simulink model "NBMS_SoC"  (R2026b)
settings: Solver=FixedStepDiscrete  StopTime=25  FixedStep=0.1
undefined symbols (not defined in the file): BMS_BattSoCDerate_E, BMS_BattTempDerate_E, BMS_MODE_E, CAL_15_SOC_WRN_RVL_THRSH, CAL_15_SOC_WRN_THRSH, CAL_DCHRG_END_THRSH, CAL_DOD, CAL_DOD_MAX_THRSH, CAL_DOD_MIN_THRSH, CAL_ENABLE_SOC_WARN_15, CAL_ENABLE_SOC_WARN_20, CAL_GOLDEN_CHARGE, CAL_GOLDEN_DC, CAL_LOW_SOC_RVL_THRSH, CAL_LOW_SOC_THRSH, CAL_NOMINAL_VOLTAGE, CAL_SOC_WRN_RVL_THRSH, CAL_SOC_WRN_THRSH, CAL_SOH_Enable, Charger_Mode_Req_E, DiscIntNeverNeededParam, OBC_E, VDU_MACHINE_STS_E, X_DCIR_CHG, X_DCIR_DISCH, Y_DCIR_CHG, Y_DCIR_DISCH
libraries: simulink x110, simulink_extras x6, sl_discontinuities x3
(part 1 of 3)
settings Model: Creator=hp  LastModifiedBy=rathi
settings OptimizationCC: DefaultParameterBehavior=Inlined  DifferentSizesBufferReuse=on  EfficientTunableParamExpr=on  EnhancedBackFolding=on  OptimizationCustomize=off  OptimizeBlockOrder=speed  PassReuseOutputArgsAs=Individual arguments  RemoveInternalMemoryZeroInit=on  RemoveRootLevelIOMemoryZeroInit=on
settings DebuggingCC: ParameterTunabilityLossMsg=error
settings SFSimCC: MATLABDynamicMemAlloc=off
settings RTWCC: Description=Embedded Coder  GenCodeOnly=on  PackageGeneratedCodeAndArtifacts=on  SystemTargetFile=ert.tlc  TemplateMakefile=ert_default_tmf
settings CodeAppCC: ForceParamTrailComments=on  IgnoreCustomStorageClasses=off  InsertBlockDesc=on  OperatorAnnotations=on  SFDataObjDesc=on  SimulinkDataObjDesc=on
settings ERTTargetCC: DynamicArrayContainerType=coder::array  GenerateSampleERTMain=on
settings ConfigComp: DVDefectChecker=on  DVDetectOutOfBounds=on  DVHarnessSource=Signal Editor  DVModelReferenceHarness=on  DVTestSuiteOptimization=Auto

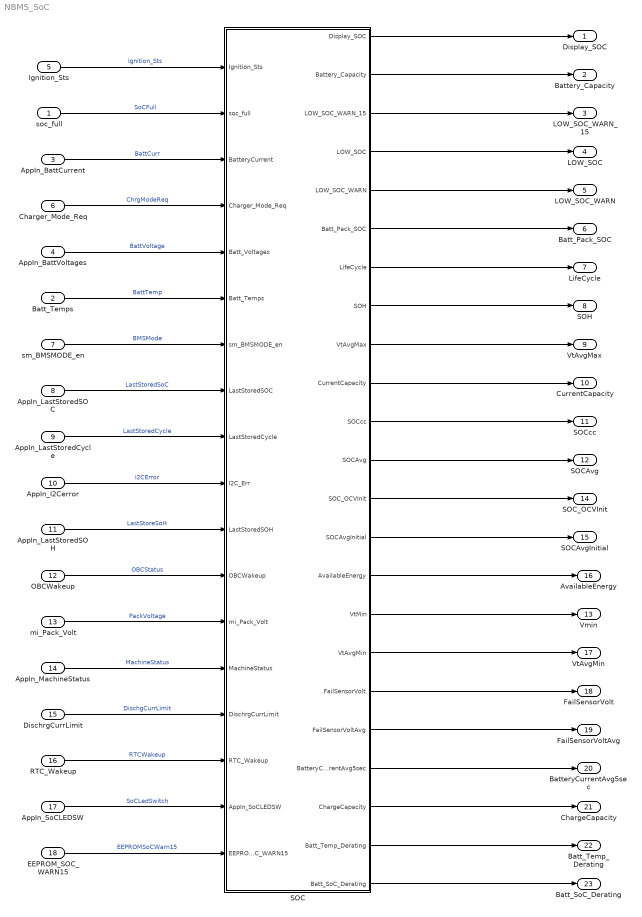
== system NBMS_SoC ==
  soc_full : Inport  OutDataTypeStr=uint8
  Batt_Temps : Inport  Port=2  OutDataTypeStr=double
  AppIn_BattCurrent : Inport  Port=3
  AppIn_BattVoltages : Inport  Port=4  OutDataTypeStr=double  PortDimensions=[20,1]
  Ignition_Sts : Inport  Port=5  OutDataTypeStr=boolean
  Charger_Mode_Req : Inport  Port=6  OutDataTypeStr=Enum:Charger_Mode_Req_E
  sm_BMSMODE_en : Inport  Port=7  OutDataTypeStr=Enum: BMS_MODE_E
  AppIn_LastStoredSOC : Inport  Port=8  OutDataTypeStr=double
  AppIn_LastStoredCycle : Inport  Port=9  OutDataTypeStr=double
  AppIn_I2Cerror : Inport  Port=10  OutDataTypeStr=boolean
  AppIn_LastStoredSOH : Inport  Port=11  OutDataTypeStr=double
  OBCWakeup : Inport  Port=12  OutDataTypeStr=Enum: OBC_E
  mi_Pack_Volt : Inport  Port=13  OutDataTypeStr=double
  AppIn_MachineStatus : Inport  Port=14  OutDataTypeStr=Enum: VDU_MACHINE_STS_E
  DischrgCurrLimit : Inport  Port=15
  RTC_Wakeup : Inport  Port=16  OutDataTypeStr=boolean
  AppIn_SoCLEDSW : Inport  Port=17  OutDataTypeStr=boolean
  EEPROM_SOC_WARN15 : Inport  Port=18  OutDataTypeStr=boolean
  SOC : Subsystem
  Display_SOC : Outport  OutDataTypeStr=uint8
  Battery_Capacity : Outport  Port=2
  LOW_SOC_WARN_15 : Outport  Port=3  OutDataTypeStr=boolean
  LOW_SOC : Outport  Port=4  OutDataTypeStr=boolean
  LOW_SOC_WARN : Outport  Port=5  OutDataTypeStr=boolean
  Batt_Pack_SOC : Outport  Port=6
  LifeCycle : Outport  Port=7  OutDataTypeStr=double
  SOH : Outport  Port=8  OutDataTypeStr=double
  VtAvgMax : Outport  Port=9  OutDataTypeStr=fixdt(1,16,0.001,0)
  CurrentCapacity : Outport  Port=10  OutDataTypeStr=double
  SOCcc : Outport  Port=11  OutDataTypeStr=fixdt(0,16,0.01,0)
  SOCAvg : Outport  Port=12  OutDataTypeStr=fixdt(0,16,0.01,0)
  Vmin : Outport  Port=13  OutDataTypeStr=fixdt(1,16,0.001,0)
  SOC_OCVInit : Outport  Port=14  OutDataTypeStr=double
  SOCAvgInitial : Outport  Port=15  OutDataTypeStr=double
  AvailableEnergy : Outport  Port=16  OutDataTypeStr=double
  VtAvgMin : Outport  Port=17
  FailSensorVolt : Outport  Port=18  OutputWhenDisabled=reset  InitialOutput=5
  FailSensorVoltAvg : Outport  Port=19  OutputWhenDisabled=reset  InitialOutput=5
  BatteryCurrentAvg5sec : Outport  Port=20  OutDataTypeStr=fixdt(1,16,0.01,0)
  ChargeCapacity : Outport  Port=21  OutDataTypeStr=double
  Batt_Temp_Derating : Outport  Port=22  OutDataTypeStr=Enum: BMS_BattTempDerate_E
  Batt_SoC_Derating : Outport  Port=23  OutDataTypeStr=Enum: BMS_BattSoCDerate_E
  wires:
  SOC/5(" LOW_SOC_WARN") -> LOW_SOC_WARN/1
  SOC/13(SOC_OCVInit) -> SOC_OCVInit/1
  SOC/17(VtAvgMin) -> VtAvgMin/1
  SOC/9(VtAvgMax) -> VtAvgMax/1
  SOC/14(SOCAvgInitial) -> SOCAvgInitial/1
  SOC/21(ChargeCapacity) -> ChargeCapacity/1
  SOC/1(Display_SOC) -> Display_SOC/1
  SOC/15(AvailableEnergy) -> AvailableEnergy/1
  AppIn_LastStoredCycle/1 -> SOC/9(LastStoredCycle)  "LastStoredCycle"
  SOC/11(SOCcc) -> SOCcc/1
  SOC/8(SOH) -> SOH/1
  OBCWakeup/1 -> SOC/12(OBCWakeup)  "OBCStatus"
  SOC/16(VtMin) -> Vmin/1
  SOC/10(CurrentCapacity) -> CurrentCapacity/1
  SOC/6(Batt_Pack_SOC) -> Batt_Pack_SOC/1
  AppIn_BattVoltages/1 -> SOC/5(Batt_Voltages)  "BattVoltage"
  SOC/12(SOCAvg) -> SOCAvg/1
  SOC/20(BatteryCurrentAvg5sec) -> BatteryCurrentAvg5sec/1
  AppIn_LastStoredSOH/1 -> SOC/11(LastStoredSOH)  "LastStoreSoH"
  SOC/7(LifeCycle) -> LifeCycle/1
  SOC/3(" LOW_SOC_WARN_15") -> LOW_SOC_WARN_15/1
  SOC/2(Battery_Capacity) -> Battery_Capacity/1
  mi_Pack_Volt/1 -> SOC/13(mi_Pack_Volt)  "PackVoltage"
  DischrgCurrLimit/1 -> SOC/15(DischrgCurrLimit)  "DischgCurrLimit"
  SOC/4(" LOW_SOC") -> LOW_SOC/1
  SOC/19(FailSensorVoltAvg) -> FailSensorVoltAvg/1
  Charger_Mode_Req/1 -> SOC/4(Charger_Mode_Req)  "ChrgModeReq"
  sm_BMSMODE_en/1 -> SOC/7(sm_BMSMODE_en)  "BMSMode"
  Batt_Temps/1 -> SOC/6(Batt_Temps)  "BattTemp"
  AppIn_MachineStatus/1 -> SOC/14(MachineStatus)  "MachineStatus"
  SOC/18(FailSensorVolt) -> FailSensorVolt/1
  AppIn_I2Cerror/1 -> SOC/10(I2C_Err)  "I2CError"
  soc_full/1 -> SOC/2(soc_full)  "SoCFull"
  AppIn_BattCurrent/1 -> SOC/3(BatteryCurrent)  "BattCurr"
  AppIn_LastStoredSOC/1 -> SOC/8(LastStoredSOC)  "LastStoredSoC"
  Ignition_Sts/1 -> SOC/1(Ignition_Sts)  "Ignition_Sts"
  SOC/22(Batt_Temp_Derating) -> Batt_Temp_Derating/1
  SOC/23(Batt_SoC_Derating) -> Batt_SoC_Derating/1
  RTC_Wakeup/1 -> SOC/16(RTC_Wakeup)  "RTCWakeup"
  AppIn_SoCLEDSW/1 -> SOC/17(AppIn_SoCLEDSW)  "SoCLedSwitch"
  EEPROM_SOC_WARN15/1 -> SOC/18(EEPROM_SOC_WARN15)  "EEPROMSoCWarn15"

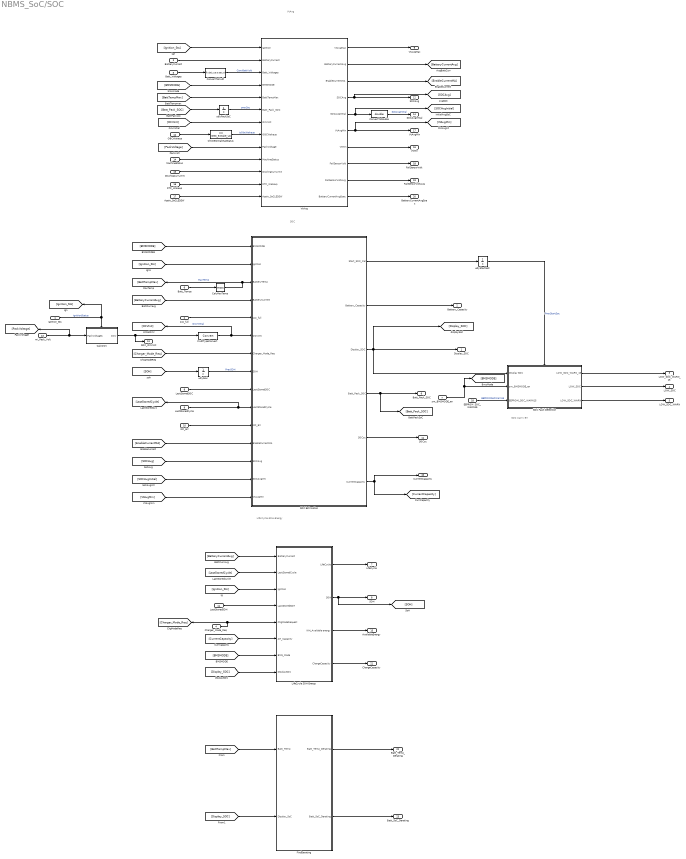
== system NBMS_SoC/SOC ==
  note: VtAvg
  note: SOC
  note: SOC warn / Err
  note: Life Cycle-SOH-Energy
  Ignition_Sts : Inport
  soc_full : Inport  Port=2
  BatteryCurrent : Inport  Port=3
  Charger_Mode_Req : Inport  Port=4
  Batt_Voltages : Inport  Port=5  PortDimensions=[20,1]
  Batt_Temps : Inport  Port=6  OutDataTypeStr=double  PortDimensions=[6,1]
  sm_BMSMODE_en : Inport  Port=7  OutDataTypeStr=Enum: BMS_MODE_E
  LastStoredSOC : Inport  Port=8
  LastStoredCycle : Inport  Port=9
  I2C_Err : Inport  Port=10
  LastStoredSOH : Inport  Port=11
  OBCWakeup : Inport  Port=12
  mi_Pack_Volt : Inport  Port=13  OutDataTypeStr=double
  MachineStatus : Inport  Port=14  OutDataTypeStr=Enum: VDU_MACHINE_STS_E
  DischrgCurrLimit : Inport  Port=15
  RTC_Wakeup : Inport  Port=16
  AppIn_SoCLEDSW : Inport  Port=17
  EEPROM_SOC_WARN15 : Inport  Port=18  OutDataTypeStr=boolean
  CalcMaxTemp : MinMax  Function=max
  CalcOCV : Subsystem  TreatAsAtomicUnit=on
  ChkOBCWakeupStatus : simulink/Logic and Bit Operations/Compare To Constant  relop===  const=OBC_E.Wake_Up  OutDataTypeStr=boolean
  ConvertToDouble : DataTypeConversion  OutDataTypeStr=double  SaturateOnIntegerOverflow=off  RndMeth=Floor
  ConvertToFixdt : DataTypeConversion  OutDataTypeStr=fixdt(1,16,0.001,0)  SaturateOnIntegerOverflow=off  RndMeth=Floor
  FindDerating : Subsystem
  FixdtTypeConvert : DataTypeConversion  SaturateOnIntegerOverflow=off  RndMeth=Floor
  LifeCycle SOH Energy : Subsystem
  SOC Estimation : Subsystem
  SOC Fault Detection : Subsystem
  VtAvg : Subsystem
  udlyPackSoC : UnitDelay  InitialCondition=1  SampleTime=-1
  udlySoH : UnitDelay  InitialCondition=1  SampleTime=-1
  udlyStartSoC : UnitDelay  SampleTime=-1
  Display_SOC : Outport
  Battery_Capacity : Outport  Port=2
  " LOW_SOC_WARN_15" : Outport  Port=3
  " LOW_SOC" : Outport  Port=4
  " LOW_SOC_WARN" : Outport  Port=5
  Batt_Pack_SOC : Outport  Port=6
  LifeCycle : Outport  Port=7
  SOH : Outport  Port=8
  VtAvgMax : Outport  Port=9
  CurrentCapacity : Outport  Port=10
  SOCcc : Outport  Port=11
  SOCAvg : Outport  Port=12
  SOC_OCVInit : Outport  Port=13
  SOCAvgInitial : Outport  Port=14
  AvailableEnergy : Outport  Port=15  OutDataTypeStr=double
  VtMin : Outport  Port=16
  VtAvgMin : Outport  Port=17
  FailSensorVolt : Outport  Port=18  OutputWhenDisabled=reset  InitialOutput=5
  FailSensorVoltAvg : Outport  Port=19  OutputWhenDisabled=reset  InitialOutput=5
  BatteryCurrentAvg5sec : Outport  Port=20  OutDataTypeStr=fixdt(1,16,0.01,0)
  ChargeCapacity : Outport  Port=21
  Batt_Temp_Derating : Outport  Port=22  OutDataTypeStr=Enum: BMS_BattTempDerate_E
  Batt_SoC_Derating : Outport  Port=23  OutDataTypeStr=Enum: BMS_BattSoCDerate_E
  wires:
  ConvertToDouble/1 -> SOCAvgInitial/1  "SoCAvgInitial"
  SOC Estimation/1(Start_SOC_Cal) -> udlyStartSoC/1
  FixdtTypeConvert/1 -> [OCVInit], SOC Estimation/6(OCVInit)  "OCVInitial"
  mi_Pack_Volt/1 -> [PackVoltage], CalcOCV/1(PackVoltages)
  [LastStoredCycle] -> LifeCycle SOH Energy/2(LastStoredCycle)
  [SOH] -> udlySoH/1
  [SOCAvgInitial] -> SOC Estimation/14(SOCAvgInit)
  VtAvg/5(SOCAvgInitial) -> [SOCAvgInitial], ConvertToDouble/1
  [SOCAvg] -> SOC Estimation/13(SOCAvg)
  [EnableCurrentMA] -> SOC Estimation/12(EnableCurrentMA)
  VtAvg/3(EnableCurrentMA) -> [EnableCurrentMA]
  [BatteryCurrentAvg] -> SOC Estimation/4(BatteryCurrent)
  [Charger_Mode_Req] -> SOC Estimation/7(Charger_Mode_Req)
  [Batt_Pack_SOC] -> udlyPackSoC/1
  [Display_SOC] -> LifeCycle SOH Energy/8(DisplaySOC)
  ConvertToFixdt/1 -> VtAvg/3(Batt_Voltages)  "ConvBattVolt"
  [BatteryCurrentAvg] -> LifeCycle SOH Energy/1(BatteryCurrent)
  [Ignition_Sts] -> LifeCycle SOH Energy/3(Ignition)
  [Ignition_Sts] -> VtAvg/1(Ignition)
  ChkOBCWakeupStatus/1 -> VtAvg/8(OBCWakeup)  "IsObcWakeup"
  OBCWakeup/1 -> ChkOBCWakeupStatus/1
  [OCVInit] -> VtAvg/7(OCVInit)
  VtAvg/4(SOCAvg) -> SOCAvg/1, [SOCAvg]
  [BattTempMax] -> VtAvg/5(BattTempMax)
  udlyPackSoC/1 -> VtAvg/6(Batt_Pack_SOC)  "prevSoc"
  [BMSMODE] -> VtAvg/4(BMSMODE)
  VtAvg/2(BatteryCurrentAvg) -> [BatteryCurrentAvg]
  SOC Estimation/5(SOCcc) -> SOCcc/1
  SOC Estimation/6(CurrentCapacity) -> CurrentCapacity/1, [CurrentCapacity]
  VtAvg/1(VtAvgMax) -> VtAvgMax/1
  Batt_Voltages/1 -> ConvertToFixdt/1
  udlyStartSoC/1 -> SOC Fault Detection/Enable  "PrevStartSoc"
  [BMSMODE] -> SOC Estimation/1(BMSMODE)
  LastStoredSOH/1 -> LifeCycle SOH Energy/4(LastStoredSOH)
  Ignition_Sts/1 -> [Ignition_Sts], CalcOCV/Trigger  "IgnitionStatus"
  udlySoH/1 -> SOC Estimation/8(SOH)  "PrevSOH"
  SOC Estimation/2(Battery_Capacity) -> Battery_Capacity/1
  LifeCycle SOH Energy/1(LifeCycle) -> LifeCycle/1
  SOC Estimation/3(Display_SOC) -> SOC Fault Detection/1(Display SOC), Display_SOC/1, [Display_SOC]
  BatteryCurrent/1 -> VtAvg/2(BatteryCurrent)
  SOC Fault Detection/3(" LOW_SOC_WARN") -> " LOW_SOC_WARN"/1
  SOC Fault Detection/2(" LOW_SOC") -> " LOW_SOC"/1
  SOC Fault Detection/1(" LOW_SOC_WARN_15") -> " LOW_SOC_WARN_15"/1
  sm_BMSMODE_en/1 -> SOC Fault Detection/2(sm_BMSMODE_en), [BMSMODE]
  I2C_Err/1 -> SOC Estimation/11(I2C_Err)
  SOC Estimation/4(Batt_Pack_SOC) -> Batt_Pack_SOC/1, [Batt_Pack_SOC]
  LastStoredCycle/1 -> [LastStoredCycle], SOC Estimation/10(LastStoredCycle)
  LastStoredSOC/1 -> SOC Estimation/9(LastStoredSOC)
  LifeCycle SOH Energy/2(SOH) -> SOH/1, [SOH]
  soc_full/1 -> SOC Estimation/5(soc_full)
  Charger_Mode_Req/1 -> LifeCycle SOH Energy/5(ChgModeRequest), [Charger_Mode_Req]
  CalcMaxTemp/1 -> [BattTempMax], SOC Estimation/3(BatteryTemp)  "MaxTemp"
  CalcOCV/1(OCV) -> SOC_OCVInit/1, FixdtTypeConvert/1
  Batt_Temps/1 -> CalcMaxTemp/1
  VtAvg/6(VtAvgMin) -> VtAvgMin/1, [VtAvgMin]
  [VtAvgMin] -> SOC Estimation/15(VtAvgMin)
  LifeCycle SOH Energy/3(WH_Available energy) -> AvailableEnergy/1
  [CurrentCapacity] -> LifeCycle SOH Energy/6(AH_Capacity)
  VtAvg/7(VtMin) -> VtMin/1
  [PackVoltage] -> VtAvg/9(PackVoltage)
  VtAvg/8(FailSensorVolt) -> FailSensorVolt/1
  VtAvg/9(FailSensorVoltAvg) -> FailSensorVoltAvg/1
  VtAvg/10(BatteryCurrentAvg5sec) -> BatteryCurrentAvg5sec/1
  [BMSMODE] -> LifeCycle SOH Energy/7(BMS_Mode)
  MachineStatus/1 -> VtAvg/10(MachineStatus)
  DischrgCurrLimit/1 -> VtAvg/11(DischrgCurrLimit)
  LifeCycle SOH Energy/4(ChargeCapacity) -> ChargeCapacity/1
  [Ignition_Sts] -> SOC Estimation/2(Ignition)
  [BattTempMax] -> FindDerating/1(Batt_Temp)
  [Display_SOC] -> FindDerating/2(Display_SoC)
  FindDerating/1(Batt_Temp_Derating) -> Batt_Temp_Derating/1
  FindDerating/2(Batt_SoC_Derating) -> Batt_SoC_Derating/1
  RTC_Wakeup/1 -> VtAvg/12(RTC_Wakeup)
  AppIn_SoCLEDSW/1 -> VtAvg/13(AppIn_SoCLEDSW)
  EEPROM_SOC_WARN15/1 -> SOC Fault Detection/3(EEPROM_SOC_WARN15)  "EEPROMSoCWarn15"

== system NBMS_SoC/SOC/CalcOCV ==
  PackVoltages : Inport
  Trigger : TriggerPort  VariantControl=(inherit)  PortDimensions=1
  CalcSingleCellVolt : Product  Inputs=*/
  TotalCellinSeries : Constant  Value=20
  OCV : Outport  InitialOutput=0
  wires:
  TotalCellinSeries/1 -> CalcSingleCellVolt/2  "CellinSeries"
  CalcSingleCellVolt/1 -> OCV/1  "InitOpenCircuitVoltage"
  PackVoltages/1 -> CalcSingleCellVolt/1  "RawBattPackVolt"

== system NBMS_SoC/SOC/FindDerating ==
  Batt_Temp : Inport  OutDataTypeStr=double
  Display_SoC : Inport  Port=2  OutDataTypeStr=uint8
  ChkSoCbelow20 : simulink/Logic and Bit Operations/Compare To Constant  relop=<=  const=20  OutDataTypeStr=boolean
  ChkTempabove56 : simulink/Logic and Bit Operations/Compare To Constant  relop=>=  const=56  OutDataTypeStr=boolean
  ChkTempbelow10 : simulink/Logic and Bit Operations/Compare To Constant  relop=<  const=10  OutDataTypeStr=boolean
  Derate : simulink/Sources/Enumerated Constant  OutDataTypeStr=Enum: BMS_BattTempDerate_E  Value=BMS_BattTempDerate_E.Temp_Derating  SampleTime=inf
  Derate1 : simulink/Sources/Enumerated Constant  OutDataTypeStr=Enum: BMS_BattTempDerate_E  Value=BMS_BattTempDerate_E.Temp_NoDerating  SampleTime=inf
  Derate2 : simulink/Sources/Enumerated Constant  OutDataTypeStr=Enum: BMS_BattSoCDerate_E  Value=BMS_BattSoCDerate_E.SOC_NoDerating  SampleTime=inf
  Derate3 : simulink/Sources/Enumerated Constant  OutDataTypeStr=Enum: BMS_BattSoCDerate_E  Value=BMS_BattSoCDerate_E.SOC_Derating  SampleTime=inf
  Isvalid : Logic  Operator=OR  AllPortsSameDT=off  OutDataTypeStr=boolean
  selderateflg : Switch  Criteria=u2 ~= 0  SaturateOnIntegerOverflow=off  InputSameDT=off
  selderateflg1 : Switch  Criteria=u2 ~= 0  SaturateOnIntegerOverflow=off  InputSameDT=off
  Batt_Temp_Derating : Outport  OutDataTypeStr=Enum: BMS_BattTempDerate_E
  Batt_SoC_Derating : Outport  Port=2  OutDataTypeStr=Enum: BMS_BattSoCDerate_E
  wires:
  Batt_Temp/1 -> ChkTempabove56/1, ChkTempbelow10/1  "Temperature"
  ChkTempbelow10/1 -> Isvalid/1  "IsTempbelow10"
  ChkTempabove56/1 -> Isvalid/2  "IsTempabove56"
  Isvalid/1 -> selderateflg/2  "validflag"
  Display_SoC/1 -> ChkSoCbelow20/1  "SoC"
  ChkSoCbelow20/1 -> selderateflg1/2  "IsSoCbelow20"
  selderateflg/1 -> Batt_Temp_Derating/1  "Batt_Temp_Derating"
  selderateflg1/1 -> Batt_SoC_Derating/1  "Batt_SoC_Derating"
  Derate/1 -> selderateflg/1  "derating"
  Derate1/1 -> selderateflg/3  "No derating"
  Derate2/1 -> selderateflg1/3  "No derating"
  Derate3/1 -> selderateflg1/1  "derating"

== system NBMS_SoC/SOC/LifeCycle SOH Energy ==
  BatteryCurrent : Inport
  LastStoredCycle : Inport  Port=2
  Ignition : Inport  Port=3
  LastStoredSOH : Inport  Port=4
  ChgModeRequest : Inport  Port=5
  AH_Capacity : Inport  Port=6  OutDataTypeStr=double
  BMS_Mode : Inport  Port=7
  DisplaySOC : Inport  Port=8
  "CalcAvailableEnergy " : Subsystem
  ConverToDouble : DataTypeConversion  OutDataTypeStr=double  SaturateOnIntegerOverflow=off  RndMeth=Floor
  Life Cycle : Subsystem
  State of Health : Subsystem
  calNominalVoltage : Constant  Value=CAL_NOMINAL_VOLTAGE
  gainNominalVt : Gain  Gain=0.001  OutDataTypeStr=double
  udlyLifeCycle : UnitDelay  SampleTime=-1
  LifeCycle : Outport
  SOH : Outport  Port=2
  WH_Available energy : Outport  Port=3  OutDataTypeStr=double
  ChargeCapacity : Outport  Port=4
  wires:
  LastStoredSOH/1 -> State of Health/6(LastStoredSOH)
  Ignition/1 -> State of Health/5(Ignition)
  Life Cycle/1(LifeCycle) -> LifeCycle/1, udlyLifeCycle/1
  udlyLifeCycle/1 -> State of Health/4(LifeCycle)  "PrevLifeCycle"
  DisplaySOC/1 -> State of Health/2(Display_SoC)
  ChgModeRequest/1 -> State of Health/3(Chrg_Mode_Req)
  LastStoredCycle/1 -> Life Cycle/1(LastStoredCycle)
  BatteryCurrent/1 -> ConverToDouble/1  "BattCurr"
  AH_Capacity/1 -> "CalcAvailableEnergy "/1(AH_Capacity)  "CapacityAh"
  "CalcAvailableEnergy "/1(kWH_Available energy) -> WH_Available energy/1
  calNominalVoltage/1 -> gainNominalVt/1  "NominalVt"
  gainNominalVt/1 -> "CalcAvailableEnergy "/2(V_Nominal_Voltage)  "scaledNominalVt"
  BMS_Mode/1 -> State of Health/7(BMS_Mode), Life Cycle/2(BMS_Mode)  "BMSMode"
  State of Health/1(SOH) -> Life Cycle/3(SOH), SOH/1
  ConverToDouble/1 -> State of Health/1(BattCurr), Life Cycle/4(BatteryCurrent)  "doubleBattCurr"
  State of Health/2(ChargeCapacity) -> ChargeCapacity/1

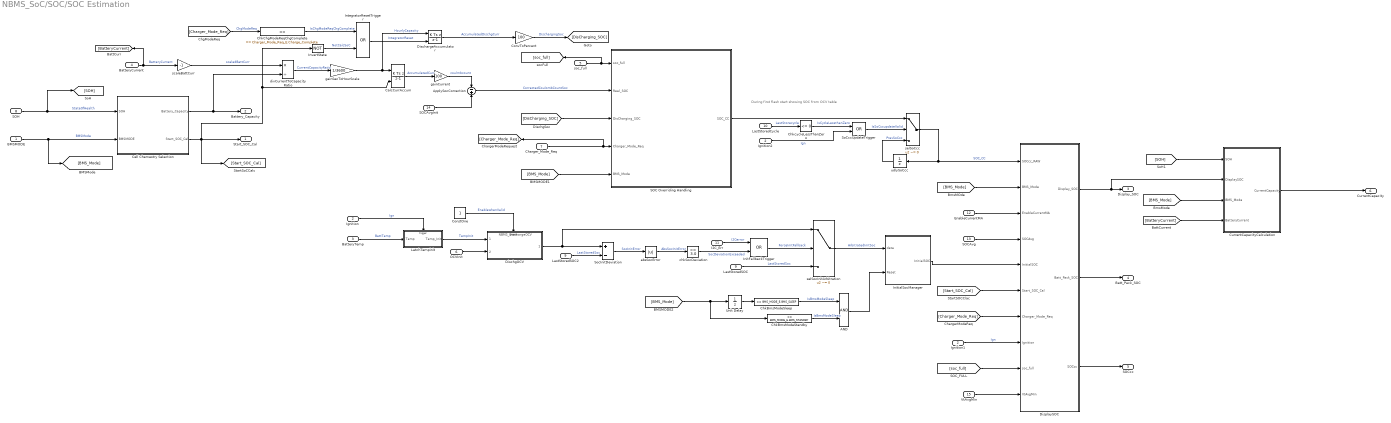
== system NBMS_SoC/SOC/SOC Estimation ==
  note: During first flash start showing SOC from OCV table
  BMSMODE : Inport
  Ignition : Inport  Port=2
  BatteryTemp : Inport  Port=3
  BatteryCurrent : Inport  Port=4
  soc_full : Inport  Port=5
  OCVInit : Inport  Port=6
  Charger_Mode_Req : Inport  Port=7
  SOH : Inport  Port=8
  LastStoredSOC : Inport  Port=9
  LastStoredCycle : Inport  Port=10
  I2C_Err : Inport  Port=11
  EnableCurrentMA : Inport  Port=12
  SOCAvg : Inport  Port=13
  SOCAvgInit : Inport  Port=14
  VtAvgMin : Inport  Port=15
  AND : Logic  AllPortsSameDT=off  OutDataTypeStr=boolean
  ApplySocCorrection : Sum  Inputs=-+
  CalcCurrAccum : DiscreteIntegrator  IntegratorMethod=Integration: Backward Euler  ExternalReset=falling  SampleTime=-1  OutDataTypeStr=double  ICPrevOutput=DiscIntNeverNeededParam  ICPrevScaledInput=DiscIntNeverNeededParam
  Cell Chemestry Selection : Subsystem
  ChkBmsModeSleep : simulink/Logic and Bit Operations/Compare To Constant  relop===  const=BMS_MODE_E.BMS_SLEEP  OutDataTypeStr=boolean
  ChkBmsModeStandby : simulink/Logic and Bit Operations/Compare To Constant  relop===  const=BMS_MODE_E.BMS_STANDBY  OutDataTypeStr=boolean
  ChkChgModeReqChgComplete : simulink/Logic and Bit Operations/Compare To Constant  relop===  const=Charger_Mode_Req_E.Charge_Complete  OutDataTypeStr=boolean
  ChkcycleLessThanZero : simulink/Logic and Bit Operations/Compare To Constant  relop=<=  const=0  OutDataTypeStr=boolean
  ConstOne : Constant  OutDataTypeStr=boolean
  ConvToPercent : Gain  Gain=100  ParamDataTypeStr=uint8
  CurrentCapacityCalculation : Subsystem
  DischargeAccumulator : DiscreteIntegrator  IntegratorMethod=Integration: Backward Euler  ExternalReset=rising  SampleTime=-1  OutDataTypeStr=double  ICPrevOutput=DiscIntNeverNeededParam  ICPrevScaledInput=DiscIntNeverNeededParam
  DischgOCV : ModelReference  ModelNameDialog=NBMS_DischargeOCV.slx  SimulationMode=Normal  ModelReferenceVersion=7.7  EnablePortName=EnableWhenValid  EnablePortStatesWhenEnabling=reset
  DisplaySOC : Subsystem
  Ignition1 : InportShadow  Port=2
  Ignition2 : InportShadow  Port=2
  InitFallbackTrigger : Logic  Operator=OR  AllPortsSameDT=off  OutDataTypeStr=boolean
  InitialSocManager : Stateflow chart  TreatAsAtomicUnit=on
  IntegratorResetTrigger : Logic  Operator=OR  AllPortsSameDT=off  OutDataTypeStr=boolean
  InvertState : Logic  Operator=NOT  AllPortsSameDT=off  OutDataTypeStr=boolean
  LastStoredSOC2 : InportShadow  Port=9
  LatchTempinit : Subsystem  TreatAsAtomicUnit=on
  SOC Overriding Handling : Subsystem
  SoCccUpdateTrigger : Logic  Operator=OR  AllPortsSameDT=off  OutDataTypeStr=boolean
  SocInitDeviation : Sum  Inputs=+-
  Unit Delay : UnitDelay  InitialCondition=BMS_MODE_E.BMS_SLEEP  SampleTime=-1
  absSocError : Abs  SaturateOnIntegerOverflow=off
  chkSocDeviation : simulink/Logic and Bit Operations/Compare To Constant  relop=>=  const=3.0  OutDataTypeStr=boolean
  divCurrentToCapacityRatio : Product  Inputs=*/
  gainCurrent : Gain  Gain=100
  gainSecToHourScale : Gain  Gain=1/3600
  scaleBattCurr : Gain  Gain=-1
  selSoCcc : Switch  Criteria=u2 ~= 0  SaturateOnIntegerOverflow=off  InputSameDT=off
  selSocInitArbitration : Switch  Criteria=u2 ~= 0  SaturateOnIntegerOverflow=off  InputSameDT=off
  udlySoCcc : UnitDelay  SampleTime=-1
  Start_SOC_Cal : Outport
  Battery_Capacity : Outport  Port=2
  Display_SOC : Outport  Port=3
  Batt_Pack_SOC : Outport  Port=4
  SOCcc : Outport  Port=5
  CurrentCapacity : Outport  Port=6
  wires:
  selSocInitArbitration/1 -> InitialSocManager/1(data)  "ArbitratedInitSoc"
  ChkBmsModeSleep/1 -> AND/1  "IsBmsModeSleep"
  DischgOCV/1 -> SocInitDeviation/1, selSocInitArbitration/1
  OCVInit/1 -> DischgOCV/2
  LastStoredSOC/1 -> selSocInitArbitration/3  "LastStoredSoc"
  InitFallbackTrigger/1 -> selSocInitArbitration/2  "ForceInitFallback"
  [soc_full] -> DisplaySOC/9(soc_full)
  [BMS_Mode] -> SOC Overriding Handling/5(BMS_Mode)
  Ignition1/1 -> DisplaySOC/8(Ignition)  "Ign"
  [Charger_Mode_Req] -> DisplaySOC/7(Charger_Mode_Req)
  [Start_SOC_Cal] -> DisplaySOC/6(Start_SOC_Cal)
  [Charger_Mode_Req] -> ChkChgModeReqChgComplete/1  "ChgModeReq"
  ChkChgModeReqChgComplete/1 -> IntegratorResetTrigger/1  "IsChgModeReqChgComplete"
  InitialSocManager/1(InitialSOC) -> DisplaySOC/5(InitialSOC)
  SOCAvgInit/1 -> ApplySocCorrection/2
  SOCAvg/1 -> DisplaySOC/4(SOCAvg)
  BatteryCurrent/1 -> scaleBattCurr/1, [BatteryCurrent]  "BatteryCurrent"
  DisplaySOC/3(SOCcc) -> SOCcc/1
  DisplaySOC/2(Batt_Pack_SOC) -> Batt_Pack_SOC/1
  EnableCurrentMA/1 -> DisplaySOC/3(EnableCurrentMA)
  [BMS_Mode] -> DisplaySOC/2(BMS_Mode)
  DisplaySOC/1(Display_SOC) -> CurrentCapacityCalculation/2(DisplaySOC), Display_SOC/1
  Cell Chemestry Selection/2(Start_SOC_Cal) -> [Start_SOC_Cal], CalcCurrAccum/2, InvertState/1, Start_SOC_Cal/1
  udlySoCcc/1 -> selSoCcc/3  "PrevSoCcc"
  SOC Overriding Handling/1(SOC_CC) -> selSoCcc/1
  SoCccUpdateTrigger/1 -> selSoCcc/2  "IsSoCccupdateValid"
  ChkcycleLessThanZero/1 -> SoCccUpdateTrigger/1  "IsCycleLessthanZero"
  LastStoredCycle/1 -> ChkcycleLessThanZero/1  "LastStorecycle"
  selSoCcc/1 -> udlySoCcc/1, DisplaySOC/1(SOCcc_RAW)  "SOC_CC"
  ApplySocCorrection/1 -> SOC Overriding Handling/2(Real_SOC)  "CorrectedCoulombCountSoc"
  gainCurrent/1 -> ApplySocCorrection/1  "coulmbcount"
  BMSMODE/1 -> [BMS_Mode], Cell Chemestry Selection/2(BMSMODE)  "BMSMode"
  IntegratorResetTrigger/1 -> DischargeAccumulator/2  "IntegratorReset"
  InvertState/1 -> IntegratorResetTrigger/2  "NotCalcSoC"
  SOH/1 -> Cell Chemestry Selection/1(SOH), [SOH]  "StateOfHealth"
  Cell Chemestry Selection/1(Battery_Capacity) -> divCurrentToCapacityRatio/2, Battery_Capacity/1
  Charger_Mode_Req/1 -> [Charger_Mode_Req], SOC Overriding Handling/4(Charger_Mode_Req)
  [DisCharging_SOC] -> SOC Overriding Handling/3(DisCharging_SOC)
  soc_full/1 -> SOC Overriding Handling/1(soc_full), [soc_full]
  DischargeAccumulator/1 -> ConvToPercent/1  "AccumulatedDischgCurr"
  ConvToPercent/1 -> [DisCharging_SOC]  "DischargingSoc"
  gainSecToHourScale/1 -> DischargeAccumulator/1, CalcCurrAccum/1  "HourlyCapacity"
  divCurrentToCapacityRatio/1 -> gainSecToHourScale/1  "CurrentCapacityRatio"
  CalcCurrAccum/1 -> gainCurrent/1  "AccumulatedCurr"
  scaleBattCurr/1 -> divCurrentToCapacityRatio/1  "scaledBattCurr"
  VtAvgMin/1 -> DisplaySOC/10(VtAvgMin)
  BatteryTemp/1 -> LatchTempinit/1(Temp)  "BattTemp"
  LatchTempinit/1(Temp_Init) -> DischgOCV/1  "TempInit"
  Ignition/1 -> LatchTempinit/Trigger  "Ign"
  I2C_Err/1 -> InitFallbackTrigger/1  "I2Cerror"
  LastStoredSOC2/1 -> SocInitDeviation/2  "LastStoredSoc"
  SocInitDeviation/1 -> absSocError/1  "SocInitError"
  absSocError/1 -> chkSocDeviation/1  "AbsSocInitError"
  chkSocDeviation/1 -> InitFallbackTrigger/2  "SocDeviationExceeded"
  ConstOne/1 -> DischgOCV/Enable  "EnablewhenValid"
  CurrentCapacityCalculation/1(CurrentCapacity) -> CurrentCapacity/1
  [SOH] -> CurrentCapacityCalculation/1(SOH)
  [BMS_Mode] -> CurrentCapacityCalculation/3(BMS_Mode)
  [BatteryCurrent] -> CurrentCapacityCalculation/4(BatteryCurrent)
  [BMS_Mode] -> ChkBmsModeStandby/1, Unit Delay/1
  Ignition2/1 -> SoCccUpdateTrigger/2  "Ign"
  AND/1 -> InitialSocManager/2(Reset)
  Unit Delay/1 -> ChkBmsModeSleep/1
  ChkBmsModeStandby/1 -> AND/2  "IsBmsModeSleep"

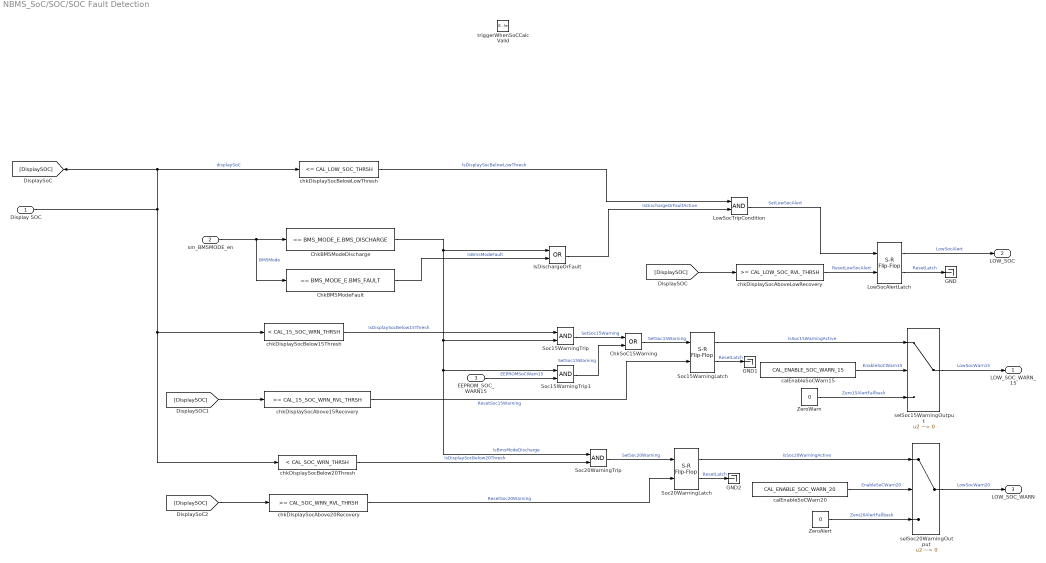
== system NBMS_SoC/SOC/SOC Fault Detection ==
  Display SOC : Inport
  sm_BMSMODE_en : Inport  Port=2  OutDataTypeStr=Enum: BMS_MODE_E
  EEPROM_SOC_WARN15 : Inport  Port=3  OutDataTypeStr=boolean
  triggerWhenSoCCalcValid : EnablePort  StatesWhenEnabling=reset
  ChkBMSModeDischarge : simulink/Logic and Bit Operations/Compare To Constant  relop===  const=BMS_MODE_E.BMS_DISCHARGE  OutDataTypeStr=boolean
  ChkBMSModeFault : simulink/Logic and Bit Operations/Compare To Constant  relop===  const=BMS_MODE_E.BMS_FAULT  OutDataTypeStr=boolean
  ChkSoC15Warning : Logic  Operator=OR  AllPortsSameDT=off  OutDataTypeStr=boolean
  GND : Terminator
  GND1 : Terminator
  GND2 : Terminator
  IsDischargeOrFault : Logic  Operator=OR  AllPortsSameDT=off  OutDataTypeStr=boolean
  LowSocAlertLatch : simulink_extras/Flip Flops/S-R Flip-Flop  initial_condition=0
  LowSocTripCondition : Logic  AllPortsSameDT=off  OutDataTypeStr=boolean
  Soc15WarningLatch : simulink_extras/Flip Flops/S-R Flip-Flop  initial_condition=0
  Soc15WarningTrip : Logic  AllPortsSameDT=off  OutDataTypeStr=boolean
  Soc15WarningTrip1 : Logic  AllPortsSameDT=off  OutDataTypeStr=boolean
  Soc20WarningLatch : simulink_extras/Flip Flops/S-R Flip-Flop  initial_condition=0
  Soc20WarningTrip : Logic  AllPortsSameDT=off  OutDataTypeStr=boolean
  ZeroAlert : Constant  Value=0  OutDataTypeStr=boolean
  ZeroWarn : Constant  Value=0  OutDataTypeStr=boolean
  calEnableSoCWarn15 : Constant  Value=CAL_ENABLE_SOC_WARN_15  OutDataTypeStr=Inherit: Inherit via back propagation
  calEnableSoCWarn20 : Constant  Value=CAL_ENABLE_SOC_WARN_20  OutDataTypeStr=Inherit: Inherit via back propagation
  chkDisplaySocAbove15Recovery : simulink/Logic and Bit Operations/Compare To Constant  relop=>=  const=CAL_15_SOC_WRN_RVL_THRSH  OutDataTypeStr=boolean
  chkDisplaySocAbove20Recovery : simulink/Logic and Bit Operations/Compare To Constant  relop=>=  const=CAL_SOC_WRN_RVL_THRSH  OutDataTypeStr=boolean
  chkDisplaySocAboveLowRecovery : simulink/Logic and Bit Operations/Compare To Constant  relop=>=  const=CAL_LOW_SOC_RVL_THRSH  OutDataTypeStr=boolean
  chkDisplaySocBelow15Thresh : simulink/Logic and Bit Operations/Compare To Constant  relop=<  const=CAL_15_SOC_WRN_THRSH  OutDataTypeStr=boolean
  chkDisplaySocBelow20Thresh : simulink/Logic and Bit Operations/Compare To Constant  relop=<  const=CAL_SOC_WRN_THRSH  OutDataTypeStr=boolean
  chkDisplaySocBelowLowThresh : simulink/Logic and Bit Operations/Compare To Constant  relop=<=  const=CAL_LOW_SOC_THRSH  OutDataTypeStr=boolean
  selSoc15WarningOutput : Switch  Criteria=u2 ~= 0  SaturateOnIntegerOverflow=off  InputSameDT=off
  selSoc20WarningOutput : Switch  Criteria=u2 ~= 0  SaturateOnIntegerOverflow=off  InputSameDT=off
  " LOW_SOC_WARN_15" : Outport  OutputWhenDisabled=reset  InitialOutput=0
  " LOW_SOC" : Outport  Port=2  OutputWhenDisabled=reset  InitialOutput=0
  " LOW_SOC_WARN" : Outport  Port=3  OutputWhenDisabled=reset  InitialOutput=0
  wires:
  ZeroAlert/1 -> selSoc20WarningOutput/3  "Zero20AlertFallback"
  calEnableSoCWarn20/1 -> selSoc20WarningOutput/2  "EnableSoCWarn20"
  Soc20WarningLatch/1 -> selSoc20WarningOutput/1  "IsSoc20WarningActive"
  selSoc20WarningOutput/1 -> " LOW_SOC_WARN"/1  "LowSocWarn20"
  selSoc15WarningOutput/1 -> " LOW_SOC_WARN_15"/1  "LowSocWarn15"
  ZeroWarn/1 -> selSoc15WarningOutput/3  "Zero15AlertFallback"
  calEnableSoCWarn15/1 -> selSoc15WarningOutput/2  "EnableSoCWarn15"
  Soc15WarningLatch/1 -> selSoc15WarningOutput/1  "IsSoc15WarningActive"
  ChkBMSModeFault/1 -> IsDischargeOrFault/2  "IsBmsModeFault"
  IsDischargeOrFault/1 -> LowSocTripCondition/2  "IsDischargeOrFaultActive"
  Soc20WarningLatch/2 -> GND2/1  "ResetLatch"
  Soc15WarningLatch/2 -> GND1/1  "ResetLatch"
  LowSocAlertLatch/2 -> GND/1  "ResetLatch"
  chkDisplaySocAbove20Recovery/1 -> Soc20WarningLatch/2  "ResetSoc20Warning"
  Soc20WarningTrip/1 -> Soc20WarningLatch/1  "SetSoc20Warning"
  [DisplaySOC] -> chkDisplaySocAbove20Recovery/1
  chkDisplaySocAbove15Recovery/1 -> Soc15WarningLatch/2  "ResetSoc15Warning"
  [DisplaySOC] -> chkDisplaySocAbove15Recovery/1
  Soc15WarningTrip/1 -> ChkSoC15Warning/1  "SetSoc15Warning"
  chkDisplaySocBelow15Thresh/1 -> Soc15WarningTrip/1  "IsDisplaySocBelow15Thresh"
  LowSocAlertLatch/1 -> " LOW_SOC"/1  "LowSocAlert"
  chkDisplaySocAboveLowRecovery/1 -> LowSocAlertLatch/2  "ResetLowSocAlert"
  [DisplaySOC] -> chkDisplaySocAboveLowRecovery/1
  LowSocTripCondition/1 -> LowSocAlertLatch/1  "SetLowSocAlert"
  ChkBMSModeDischarge/1 -> IsDischargeOrFault/1, Soc15WarningTrip/2, Soc15WarningTrip1/1, Soc20WarningTrip/1  "IsBmsModeDischarge"
  chkDisplaySocBelowLowThresh/1 -> LowSocTripCondition/1  "IsDisplaySocBelowLowThresh"
  Display SOC/1 -> [DisplaySOC], chkDisplaySocBelowLowThresh/1, chkDisplaySocBelow20Thresh/1, chkDisplaySocBelow15Thresh/1  "displaySoC"
  sm_BMSMODE_en/1 -> ChkBMSModeDischarge/1, ChkBMSModeFault/1  "BMSMode"
  chkDisplaySocBelow20Thresh/1 -> Soc20WarningTrip/2  "IsDisplaySocBelow20Thresh"
  EEPROM_SOC_WARN15/1 -> Soc15WarningTrip1/2  "EEPROMSoCWarn15"
  Soc15WarningTrip1/1 -> ChkSoC15Warning/2  "SetSoc15Warning"
  ChkSoC15Warning/1 -> Soc15WarningLatch/1  "SetSoc15Warning"

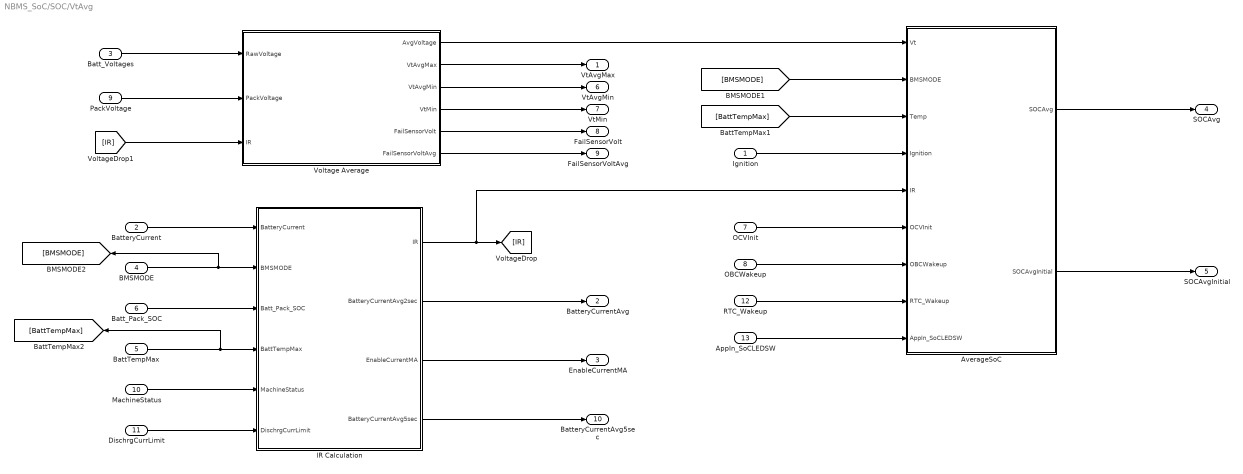
== system NBMS_SoC/SOC/VtAvg ==
  Ignition : Inport
  BatteryCurrent : Inport  Port=2
  Batt_Voltages : Inport  Port=3
  BMSMODE : Inport  Port=4
  BattTempMax : Inport  Port=5  OutDataTypeStr=double
  Batt_Pack_SOC : Inport  Port=6
  OCVInit : Inport  Port=7
  OBCWakeup : Inport  Port=8
  PackVoltage : Inport  Port=9
  MachineStatus : Inport  Port=10  OutDataTypeStr=Enum: VDU_MACHINE_STS_E
  DischrgCurrLimit : Inport  Port=11
  RTC_Wakeup : Inport  Port=12
  AppIn_SoCLEDSW : Inport  Port=13
  AverageSoC : Subsystem
  IR Calculation : Subsystem
  Voltage Average : Subsystem
  VtAvgMax : Outport
  BatteryCurrentAvg : Outport  Port=2  OutDataTypeStr=fixdt(1,16,0.01,0)
  EnableCurrentMA : Outport  Port=3  OutDataTypeStr=boolean
  SOCAvg : Outport  Port=4
  SOCAvgInitial : Outport  Port=5
  VtAvgMin : Outport  Port=6
  VtMin : Outport  Port=7
  FailSensorVolt : Outport  Port=8  OutputWhenDisabled=reset  InitialOutput=5
  FailSensorVoltAvg : Outport  Port=9  OutputWhenDisabled=reset  InitialOutput=5
  BatteryCurrentAvg5sec : Outport  Port=10  OutDataTypeStr=fixdt(1,16,0.01,0)
  wires:
  Voltage Average/1(AvgVoltage) -> AverageSoC/1(Vt)
  AverageSoC/2(SOCAvgInitial) -> SOCAvgInitial/1
  AverageSoC/1(SOCAvg) -> SOCAvg/1
  OBCWakeup/1 -> AverageSoC/7(OBCWakeup)
  OCVInit/1 -> AverageSoC/6(OCVInit)
  IR Calculation/1(IR) -> AverageSoC/5(IR), [IR]
  Ignition/1 -> AverageSoC/4(Ignition)
  [BattTempMax] -> AverageSoC/3(Temp)
  [BMSMODE] -> AverageSoC/2(BMSMODE)
  IR Calculation/3(EnableCurrentMA) -> EnableCurrentMA/1
  IR Calculation/2(BatteryCurrentAvg2sec) -> BatteryCurrentAvg/1
  Batt_Pack_SOC/1 -> IR Calculation/3(Batt_Pack_SOC)
  BattTempMax/1 -> [BattTempMax], IR Calculation/4(BattTempMax)
  BMSMODE/1 -> [BMSMODE], IR Calculation/2(BMSMODE)
  BatteryCurrent/1 -> IR Calculation/1(BatteryCurrent)
  Batt_Voltages/1 -> Voltage Average/1(RawVoltage)
  Voltage Average/2(VtAvgMax) -> VtAvgMax/1
  [IR] -> Voltage Average/3(IR)
  Voltage Average/3(VtAvgMin) -> VtAvgMin/1
  Voltage Average/4(VtMin) -> VtMin/1
  PackVoltage/1 -> Voltage Average/2(PackVoltage)
  Voltage Average/5(FailSensorVolt) -> FailSensorVolt/1
  Voltage Average/6(FailSensorVoltAvg) -> FailSensorVoltAvg/1
  IR Calculation/4(BatteryCurrentAvg5sec) -> BatteryCurrentAvg5sec/1
  MachineStatus/1 -> IR Calculation/5(MachineStatus)
  DischrgCurrLimit/1 -> IR Calculation/6(DischrgCurrLimit)
  RTC_Wakeup/1 -> AverageSoC/8(RTC_Wakeup)
  AppIn_SoCLEDSW/1 -> AverageSoC/9(AppIn_SoCLEDSW)

== system NBMS_SoC/SOC/LifeCycle SOH Energy/CalcAvailableEnergy  ==
  note: Available_energy(Wh) == Capacity(Ah) * Nominal_voltage(V)
  AH_Capacity : Inport  OutDataTypeStr=double
  V_Nominal_Voltage : Inport  Port=2  OutDataTypeStr=double
  CalcAvailEneregy : Product  OutDataTypeStr=double
  scaleAvailEnergykWh : Gain  Gain=1/1000  OutDataTypeStr=double
  kWH_Available energy : Outport  OutDataTypeStr=double
  wires:
  V_Nominal_Voltage/1 -> CalcAvailEneregy/2  "NominalVoltage"
  scaleAvailEnergykWh/1 -> kWH_Available energy/1  "AvailableEnergykWh"
  AH_Capacity/1 -> CalcAvailEneregy/1  "CurrentCapacityAH"
  CalcAvailEneregy/1 -> scaleAvailEnergykWh/1  "AvailableEnergyWh"

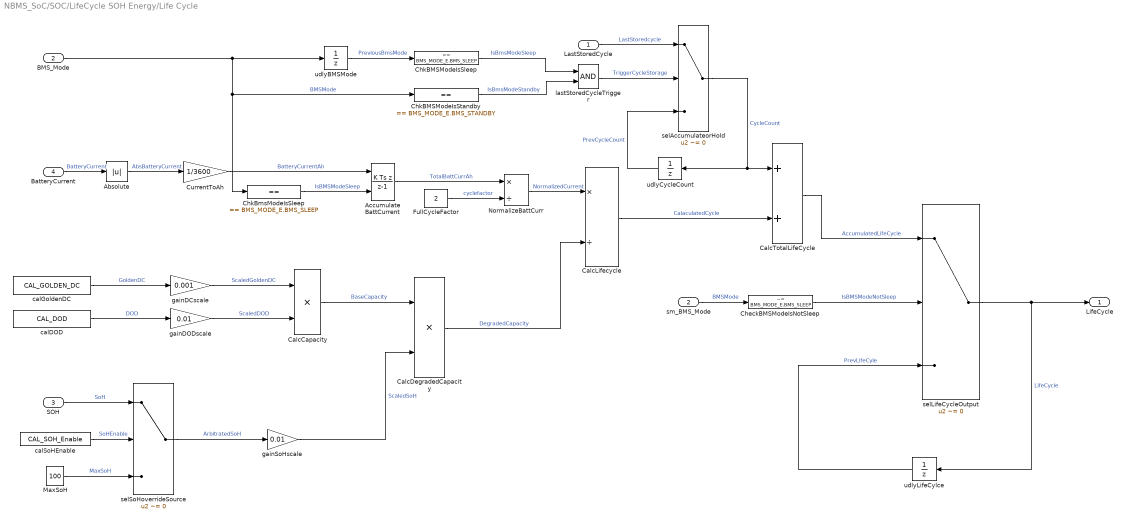
== system NBMS_SoC/SOC/LifeCycle SOH Energy/Life Cycle ==
  LastStoredCycle : Inport
  BMS_Mode : Inport  Port=2
  SOH : Inport  Port=3
  BatteryCurrent : Inport  Port=4
  Absolute : Abs  SaturateOnIntegerOverflow=off
  Accumulate BattCurrent : DiscreteIntegrator  IntegratorMethod=Integration: Backward Euler  ExternalReset=rising  SampleTime=-1  OutDataTypeStr=double  ICPrevOutput=DiscIntNeverNeededParam  ICPrevScaledInput=DiscIntNeverNeededParam
  CalcCapacity : Product  Inputs=**
  CalcDegradedCapacity : Product  Inputs=**
  CalcLifecycle : Product  Inputs=*/
  CalcTotalLifeCycle : Sum  RndMeth=Nearest
  CheckBMSModeIsNotSleep : simulink/Logic and Bit Operations/Compare To Constant  relop=~=  const=BMS_MODE_E.BMS_SLEEP  OutDataTypeStr=boolean
  ChkBMSModeIsSleep : simulink/Logic and Bit Operations/Compare To Constant  relop===  const=BMS_MODE_E.BMS_SLEEP  OutDataTypeStr=boolean
  ChkBMSModeIsStandby : simulink/Logic and Bit Operations/Compare To Constant  relop===  const=BMS_MODE_E.BMS_STANDBY  OutDataTypeStr=boolean
  ChkBmsModeIsSleep : simulink/Logic and Bit Operations/Compare To Constant  relop===  const=BMS_MODE_E.BMS_SLEEP  OutDataTypeStr=boolean
  CurrentToAh : Gain  Gain=1/3600
  FullCycleFactor : Constant  Value=2  OutDataTypeStr=Inherit: Inherit via back propagation
  MaxSoH : Constant  Value=100
  NormalizeBattCurr : Product  Inputs=*/
  calDOD : Constant  Value=CAL_DOD
  calGoldenDC : Constant  Value=CAL_GOLDEN_DC
  calSoHEnable : Constant  Value=CAL_SOH_Enable  OutDataTypeStr=Inherit: Inherit via back propagation
  gainDCscale : Gain  Gain=0.001  OutDataTypeStr=double
  gainDODscale : Gain  Gain=0.01  OutDataTypeStr=double  RndMeth=Convergent
  gainSoHscale : Gain  Gain=0.01  OutDataTypeStr=double  RndMeth=Convergent
  lastStoredCycleTrigger : Logic  AllPortsSameDT=off  OutDataTypeStr=boolean
  selAccumulateorHold : Switch  Criteria=u2 ~= 0  SaturateOnIntegerOverflow=off  InputSameDT=off
  selLifeCycleOutput : Switch  Criteria=u2 ~= 0  SaturateOnIntegerOverflow=off  InputSameDT=off
  selSoHoverrideSource : Switch  Criteria=u2 ~= 0  SaturateOnIntegerOverflow=off  InputSameDT=off
  sm_BMS_Mode : InportShadow  Port=2
  udlyBMSMode : UnitDelay  InitialCondition=BMS_MODE_E.BMS_SLEEP  SampleTime=-1
  udlyCycleCount : UnitDelay  SampleTime=-1
  udlyLifeCylce : UnitDelay  SampleTime=-1
  LifeCycle : Outport
  wires:
  MaxSoH/1 -> selSoHoverrideSource/3  "MaxSoH"
  SOH/1 -> selSoHoverrideSource/1  "SoH"
  calSoHEnable/1 -> selSoHoverrideSource/2  "SoHEnable"
  calDOD/1 -> gainDODscale/1  "DOD"
  calGoldenDC/1 -> gainDCscale/1  "GoldenDC"
  selSoHoverrideSource/1 -> gainSoHscale/1  "ArbitratedSoH"
  LastStoredCycle/1 -> selAccumulateorHold/1  "LastStoredcycle"
  BatteryCurrent/1 -> Absolute/1  "BatteryCurrent"
  sm_BMS_Mode/1 -> CheckBMSModeIsNotSleep/1  "BMSMode"
  Absolute/1 -> CurrentToAh/1  "AbsBatteryCurrent"
  CurrentToAh/1 -> Accumulate BattCurrent/1  "BatteryCurrentAh"
  Accumulate BattCurrent/1 -> NormalizeBattCurr/1  "TotalBattCurrAh"
  FullCycleFactor/1 -> NormalizeBattCurr/2  "cyclefactor"
  NormalizeBattCurr/1 -> CalcLifecycle/1  "NormalizedCurrent"
  CalcDegradedCapacity/1 -> CalcLifecycle/2  "DegradedCapacity"
  CalcCapacity/1 -> CalcDegradedCapacity/1  "BaseCapacity"
  gainSoHscale/1 -> CalcDegradedCapacity/2  "ScaledSoH"
  gainDCscale/1 -> CalcCapacity/1  "ScaledGoldenDC"
  gainDODscale/1 -> CalcCapacity/2  "ScaledDOD"
  ChkBmsModeIsSleep/1 -> Accumulate BattCurrent/2  "IsBMSModeSleep"
  CalcLifecycle/1 -> CalcTotalLifeCycle/2  "CalaculatedCycle"
  selAccumulateorHold/1 -> udlyCycleCount/1, CalcTotalLifeCycle/1  "CycleCount"
  udlyCycleCount/1 -> selAccumulateorHold/3  "PrevCycleCount"
  lastStoredCycleTrigger/1 -> selAccumulateorHold/2  "TriggerCycleStorage"
  ChkBMSModeIsSleep/1 -> lastStoredCycleTrigger/1  "IsBmsModeSleep"
  ChkBMSModeIsStandby/1 -> lastStoredCycleTrigger/2  "IsBmsModeStandby"
  udlyBMSMode/1 -> ChkBMSModeIsSleep/1  "PreviousBmsMode"
  selLifeCycleOutput/1 -> udlyLifeCylce/1, LifeCycle/1  "LifeCycle"
  CalcTotalLifeCycle/1 -> selLifeCycleOutput/1  "AccumulatedLifeCycle"
  CheckBMSModeIsNotSleep/1 -> selLifeCycleOutput/2  "IsBMSModeNotSleep"
  udlyLifeCylce/1 -> selLifeCycleOutput/3  "PrevLifeCyle"
  BMS_Mode/1 -> udlyBMSMode/1, ChkBMSModeIsStandby/1, ChkBmsModeIsSleep/1  "BMSMode"

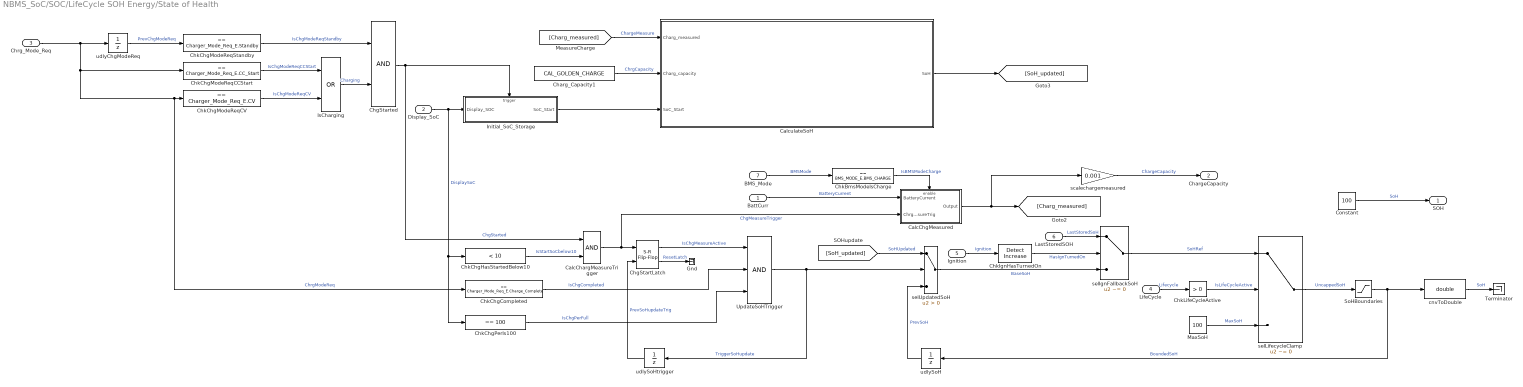
== system NBMS_SoC/SOC/LifeCycle SOH Energy/State of Health ==
  BattCurr : Inport  OutDataTypeStr=double
  Display_SoC : Inport  Port=2  OutDataTypeStr=uint8
  Chrg_Mode_Req : Inport  Port=3  OutDataTypeStr=Enum: Charger_Mode_Req_E
  LifeCycle : Inport  Port=4
  Ignition : Inport  Port=5
  LastStoredSOH : Inport  Port=6
  BMS_Mode : Inport  Port=7
  CalcChargMeasureTrigger : Logic  AllPortsSameDT=off  OutDataTypeStr=boolean
  CalcChgMeasured : Subsystem  TreatAsAtomicUnit=on
  CalculateSoH : Subsystem
  Charg_Capacity1 : Constant  Value=CAL_GOLDEN_CHARGE
  ChgStartLatch : simulink_extras/Flip Flops/S-R Flip-Flop  initial_condition=0
  ChgStarted : Logic  AllPortsSameDT=off  OutDataTypeStr=boolean
  ChkBmsModeIsCharge : simulink/Logic and Bit Operations/Compare To Constant  relop===  const=BMS_MODE_E.BMS_CHARGE  OutDataTypeStr=boolean
  ChkChgCompleted : simulink/Logic and Bit Operations/Compare To Constant  relop===  const=Charger_Mode_Req_E.Charge_Complete  OutDataTypeStr=boolean
  ChkChgHasStartedBelow10 : simulink/Logic and Bit Operations/Compare To Constant  relop=<  const=10  OutDataTypeStr=boolean
  ChkChgModeReqCCStart : simulink/Logic and Bit Operations/Compare To Constant  relop===  const=Charger_Mode_Req_E.CC_Start  OutDataTypeStr=boolean
  ChkChgModeReqCV : simulink/Logic and Bit Operations/Compare To Constant  relop===  const=Charger_Mode_Req_E.CV  OutDataTypeStr=boolean
  ChkChgModeReqStandby : simulink/Logic and Bit Operations/Compare To Constant  relop===  const=Charger_Mode_Req_E.Standby  OutDataTypeStr=boolean
  ChkChgPerIs100 : simulink/Logic and Bit Operations/Compare To Constant  relop===  const=100  OutDataTypeStr=boolean
  ChkIgnHasTurnedOn : simulink/Logic and Bit Operations/Detect Increase  vinit=0.0  OutDataTypeStr=boolean
  ChkLifeCycleActive : simulink/Logic and Bit Operations/Compare To Constant  relop=>  const=0  OutDataTypeStr=boolean
  Constant : Constant  Value=100  OutDataTypeStr=double
  Gnd : Terminator
  Initial_SoC_Storage : Subsystem  TreatAsAtomicUnit=on
  IsCharging : Logic  Operator=OR  AllPortsSameDT=off  OutDataTypeStr=boolean
  MaxSoH : Constant  Value=100
  SoHBoundaries : Saturate  UpperLimit=100  LowerLimit=0  OutDataTypeStr=uint8  RndMeth=Ceiling
  Terminator : Terminator
  UpdateSoHTrigger : Logic  Inputs=3  AllPortsSameDT=off  OutDataTypeStr=boolean
  cnvToDouble : DataTypeConversion  OutDataTypeStr=double  SaturateOnIntegerOverflow=off  RndMeth=Floor
  scalechargemeasured : Gain  Gain=0.001
  selIgnFallbackSoH : Switch  Criteria=u2 ~= 0  SaturateOnIntegerOverflow=off  InputSameDT=off
  selLifecycleClamp : Switch  Criteria=u2 ~= 0  Threshold=1  SaturateOnIntegerOverflow=off  InputSameDT=off
  selUpdatedSoH : Switch  Criteria=u2 > Threshold  SaturateOnIntegerOverflow=off  InputSameDT=off
  udlyChgModeReq : UnitDelay  InitialCondition=Charger_Mode_Req_E.Disabled  SampleTime=-1
  udlySoH : UnitDelay  InitialCondition=100  SampleTime=-1
  udlySoHtrigger : UnitDelay  SampleTime=-1
  SOH : Outport
  ChargeCapacity : Outport  Port=2
  wires:
  BattCurr/1 -> CalcChgMeasured/1(BatteryCurrent)  "BatteryCurrent"
  CalcChgMeasured/1(Output) -> scalechargemeasured/1, [Charg_measured]
  ChkChgModeReqCV/1 -> IsCharging/2  "IsChgModeReqCV"
  CalculateSoH/1(SoH) -> [SoH_updated]
  [Charg_measured] -> CalculateSoH/1(Charg_measured)  "ChargeMeasure"
  Chrg_Mode_Req/1 -> ChkChgCompleted/1, ChkChgModeReqCV/1, ChkChgModeReqCCStart/1, udlyChgModeReq/1  "ChrgModeReq"
  Display_SoC/1 -> Initial_SoC_Storage/1(Display_SOC), ChkChgHasStartedBelow10/1, ChkChgPerIs100/1  "DisplaySoC"
  ChkBmsModeIsCharge/1 -> CalcChgMeasured/Enable  "IsBMSModeCharge"
  UpdateSoHTrigger/1 -> selUpdatedSoH/2, udlySoHtrigger/1  "TriggerSoHupdate"
  Initial_SoC_Storage/1(SoC_Start) -> CalculateSoH/3(SoC_Start)
  ChkChgModeReqStandby/1 -> ChgStarted/1  "IsChgModeReqStandby"
  ChgStarted/1 -> CalcChargMeasureTrigger/1, Initial_SoC_Storage/Trigger  "ChgStarted"
  ChgStartLatch/2 -> Gnd/1  "ResetLatch"
  ChkChgModeReqCCStart/1 -> IsCharging/1  "IsChgModeReqCCStart"
  udlySoH/1 -> selUpdatedSoH/3  "PrevSoH"
  CalcChargMeasureTrigger/1 -> CalcChgMeasured/2(ChrgMeasureTrig), ChgStartLatch/1  "ChgMeasureTrigger"
  [SoH_updated] -> selUpdatedSoH/1  "SoHUpdated"
  ChgStartLatch/1 -> UpdateSoHTrigger/1  "IsChgMeasureActive"
  Charg_Capacity1/1 -> CalculateSoH/2(Charg_capacity)  "ChrgCapacity"
  IsCharging/1 -> ChgStarted/2  "Charging"
  udlySoHtrigger/1 -> ChgStartLatch/2  "PrevSoHupdateTrig"
  ChkChgCompleted/1 -> UpdateSoHTrigger/2  "IsChgCompleted"
  selIgnFallbackSoH/1 -> selLifecycleClamp/1  "SoHRef"
  ChkLifeCycleActive/1 -> selLifecycleClamp/2  "IsLifeCycleActive"
  ChkIgnHasTurnedOn/1 -> selIgnFallbackSoH/2  "HasIgnTurnedOn"
  LifeCycle/1 -> ChkLifeCycleActive/1  "Lifecycle"
  MaxSoH/1 -> selLifecycleClamp/3  "MaxSoH"
  LastStoredSOH/1 -> selIgnFallbackSoH/1  "LastStoredSoH"
  selUpdatedSoH/1 -> selIgnFallbackSoH/3  "BaseSoH"
  Ignition/1 -> ChkIgnHasTurnedOn/1  "Ignition"
  selLifecycleClamp/1 -> SoHBoundaries/1  "UncappedSoH"
  BMS_Mode/1 -> ChkBmsModeIsCharge/1  "BMSMode"
  SoHBoundaries/1 -> cnvToDouble/1, udlySoH/1  "BoundedSoH"
  ChkChgPerIs100/1 -> UpdateSoHTrigger/3  "IsChgPerFull"
  udlyChgModeReq/1 -> ChkChgModeReqStandby/1  "PrevChgModeReq"
  ChkChgHasStartedBelow10/1 -> CalcChargMeasureTrigger/2  "IsStartSoCbelow10"
  Constant/1 -> SOH/1  "SoH"
  scalechargemeasured/1 -> ChargeCapacity/1  "ChargeCapacity"
  cnvToDouble/1 -> Terminator/1  "SoH"

== system NBMS_SoC/SOC/SOC Estimation/Cell Chemestry Selection ==
  SOH : Inport
  BMSMODE : Inport  Port=2
  CalDOD : Constant  Value=CAL_DOD
  CalGoldenDC : Constant  Value=CAL_GOLDEN_DC
  CalSoHEnable : Constant  Value=CAL_SOH_Enable  OutDataTypeStr=Inherit: Inherit via back propagation
  CalcActualCapacity : Product
  CalcCapacity : Product
  ChkBMSModeNotSleep : simulink/Logic and Bit Operations/Compare To Constant  relop=~=  const=BMS_MODE_E.BMS_SLEEP  OutDataTypeStr=boolean
  gainDCscale : Gain  Gain=0.001  OutDataTypeStr=double  RndMeth=Convergent
  gainDODscale : Gain  Gain=0.01  OutDataTypeStr=double  RndMeth=Convergent
  selBatteryCapacitySource : Switch  Criteria=u2 ~= 0  SaturateOnIntegerOverflow=off  InputSameDT=off
  Battery_Capacity : Outport
  Start_SOC_Cal : Outport  Port=2
  wires:
  CalDOD/1 -> gainDODscale/1  "CalDOD"
  CalGoldenDC/1 -> gainDCscale/1  "CalGoldenDC"
  ChkBMSModeNotSleep/1 -> Start_SOC_Cal/1  "StartSoCCalc"
  BMSMODE/1 -> ChkBMSModeNotSleep/1  "BMSMODE"
  CalcCapacity/1 -> CalcActualCapacity/2, selBatteryCapacitySource/3  "BaseCapacity"
  CalcActualCapacity/1 -> selBatteryCapacitySource/1  "SoHcorrectedCapacity"
  selBatteryCapacitySource/1 -> Battery_Capacity/1  "BatteryCapacity"
  CalSoHEnable/1 -> selBatteryCapacitySource/2  "SoHEnable"
  SOH/1 -> CalcActualCapacity/1  "SoH"
  gainDCscale/1 -> CalcCapacity/1  "ScaledGoldenDC"
  gainDODscale/1 -> CalcCapacity/2  "ScaledDOD"

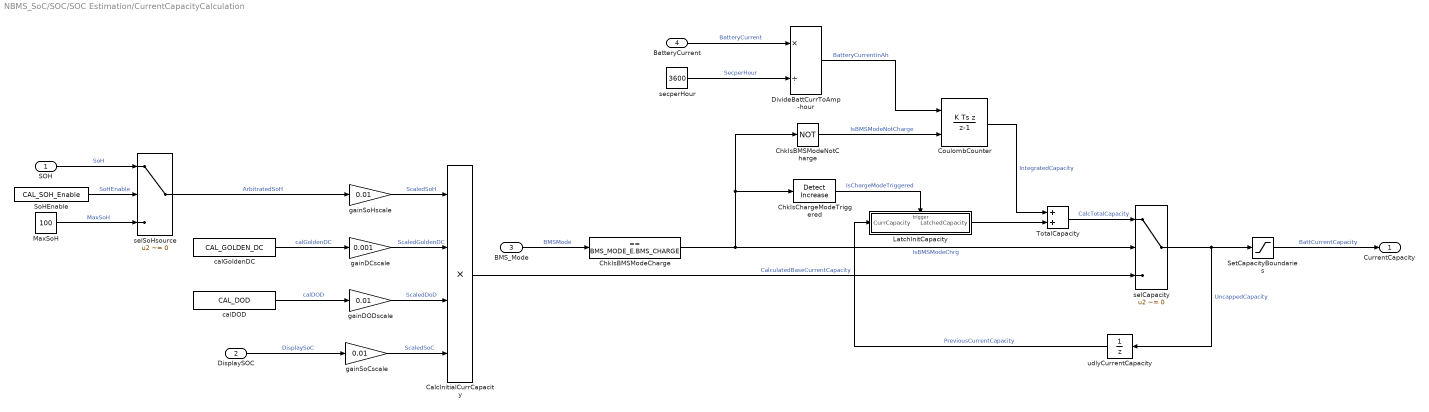
== system NBMS_SoC/SOC/SOC Estimation/CurrentCapacityCalculation ==
  SOH : Inport
  DisplaySOC : Inport  Port=2
  BMS_Mode : Inport  Port=3
  BatteryCurrent : Inport  Port=4
  CalcInitialCurrCapacity : Product  Inputs=4
  ChkIsBMSModeCharge : simulink/Logic and Bit Operations/Compare To Constant  relop===  const=BMS_MODE_E.BMS_CHARGE  OutDataTypeStr=boolean
  ChkIsBMSModeNotCharge : Logic  Operator=NOT  AllPortsSameDT=off  OutDataTypeStr=boolean
  ChkIsChargeModeTriggered : simulink/Logic and Bit Operations/Detect Increase  vinit=0.0  OutDataTypeStr=boolean
  CoulombCounter : DiscreteIntegrator  IntegratorMethod=Integration: Backward Euler  ExternalReset=rising  SampleTime=-1  OutDataTypeStr=double  LimitOutput=on  UpperSaturationLimit=38.4  LowerSaturationLimit=-38.4  ICPrevOutput=DiscIntNeverNeededParam  ICPrevScaledInput=DiscIntNeverNeededParam
  DivideBattCurrToAmp-hour : Product  Inputs=*/
  LatchInitCapacity : Subsystem  TreatAsAtomicUnit=on
  MaxSoH : Constant  Value=100
  SetCapacityBoundaries : Saturate  UpperLimit=38.4  LowerLimit=0
  SoHEnable : Constant  Value=CAL_SOH_Enable  OutDataTypeStr=Inherit: Inherit via back propagation
  TotalCapacity : Sum
  calDOD : Constant  Value=CAL_DOD
  calGoldenDC : Constant  Value=CAL_GOLDEN_DC
  gainDCscale : Gain  Gain=0.001  OutDataTypeStr=double  RndMeth=Convergent
  gainDODscale : Gain  Gain=0.01  OutDataTypeStr=double  RndMeth=Convergent
  gainSoCscale : Gain  Gain=0.01  OutDataTypeStr=double  RndMeth=Convergent
  gainSoHscale : Gain  Gain=0.01  OutDataTypeStr=double  RndMeth=Convergent
  secperHour : Constant  Value=3600
  selCapacity : Switch  Criteria=u2 ~= 0  SaturateOnIntegerOverflow=off  InputSameDT=off
  selSoHsource : Switch  Criteria=u2 ~= 0  SaturateOnIntegerOverflow=off  InputSameDT=off
  udlyCurrentCapacity : UnitDelay  SampleTime=-1
  CurrentCapacity : Outport
  wires:
  calGoldenDC/1 -> gainDCscale/1  "calGoldenDC"
  calDOD/1 -> gainDODscale/1  "calDOD"
  DisplaySOC/1 -> gainSoCscale/1  "DisplaySoC"
  BMS_Mode/1 -> ChkIsBMSModeCharge/1  "BMSMode"
  BatteryCurrent/1 -> DivideBattCurrToAmp-hour/1  "BatteryCurrent"
  secperHour/1 -> DivideBattCurrToAmp-hour/2  "SecperHour"
  DivideBattCurrToAmp-hour/1 -> CoulombCounter/1  "BatteryCurrentinAh"
  ChkIsBMSModeNotCharge/1 -> CoulombCounter/2  "IsBMSModeNotCharge"
  ChkIsBMSModeCharge/1 -> selCapacity/2, ChkIsBMSModeNotCharge/1, ChkIsChargeModeTriggered/1  "IsBMSModeChrg"
  CoulombCounter/1 -> TotalCapacity/1  "IntegratedCapacity"
  gainDCscale/1 -> CalcInitialCurrCapacity/2  "ScaledGoldenDC"
  gainDODscale/1 -> CalcInitialCurrCapacity/3  "ScaledDoD"
  gainSoCscale/1 -> CalcInitialCurrCapacity/4  "ScaledSoC"
  CalcInitialCurrCapacity/1 -> selCapacity/3  "CalculatedBaseCurrentCapacity"
  selCapacity/1 -> udlyCurrentCapacity/1, SetCapacityBoundaries/1  "UncappedCapacity"
  SetCapacityBoundaries/1 -> CurrentCapacity/1  "BattCurrentCapacity"
  TotalCapacity/1 -> selCapacity/1  "CalcTotalCapacity"
  LatchInitCapacity/1(LatchedCapacity) -> TotalCapacity/2
  udlyCurrentCapacity/1 -> LatchInitCapacity/1(CurrCapacity)  "PreviousCurrentCapacity"
  ChkIsChargeModeTriggered/1 -> LatchInitCapacity/Trigger  "IsChargeModeTriggered"
  gainSoHscale/1 -> CalcInitialCurrCapacity/1  "ScaledSoH"
  SoHEnable/1 -> selSoHsource/2  "SoHEnable"
  SOH/1 -> selSoHsource/1  "SoH"
  selSoHsource/1 -> gainSoHscale/1  "ArbitratedSoH"
  MaxSoH/1 -> selSoHsource/3  "MaxSoH"
